simulink model "commhdlQPSKTxRxLoopback"  (R2025b)
settings: Solver=FixedStepDiscrete  StartTime=0.0  StopTime=stopTime  RelTol=1e-3
PostLoadFcn:
  | hScopeConfig = get_param([gcs '/Receiver/QPSK Rx/Frequency and Time Synchronizer/Symbol Synchronizer/No HDL/QPSK Receiver Eye Diagram'],'ScopeConfiguration');
  | 
  | hScopeConfig.OpenAtSimulationStart = false;
  | hScopeConfig.Visible = false;
  | SamplesPerSymbol = 4;
  | %UpsamplesRx = 1;
  | clear hScopeConfig
InitFcn:
  | commhdlQPSKTxRxModelInit;
  | % Rate bridge: ADRV9002/Jupiter radio runs at 15.36 MHz = 2x the 7.68 MHz
  | % (4 samples/symbol @ Rsym=1.92 MHz) the QPSK Rx requires. The deployed
  | % Receiver must downsample the ADC stream by 2. UpsamplesRx=1 fed the QPSK
  | % Rx 8 sps (2x-upsampled) and broke symbol sync / the loopback bit check.
  | UpsamplesRx = 1;   %% T8 RATE FIX: rail 15.36e6 == ADC bus rate,
  | %% no ingress decimation (was 2 when the rail sat on the 7.68e6 rung)
  | UpsamplesTx = 1;
  | clear simTimingOffset;
StopFcn:
  | if exist('simTimingOffset','var')
  |   disp('Simulation completed');
  |   %QPSKTxRxVerification;
  | end
undefined symbols (not defined in the file or in its folder): Add, Config, fsym, randsrc, RandStream, Rsym, Shift
libraries: hdlsllib x141, simulink x43, dspsigops x34, dsphdlfiltering2 x6, dsphdlsigops2 x4, dsphdlmathfun2 x4, commdigbbndpm3 x4, dspmlti4 x2, commchan3 x1, commrflib2 x1, commcnvcod2 x1
(part 2 of 8)

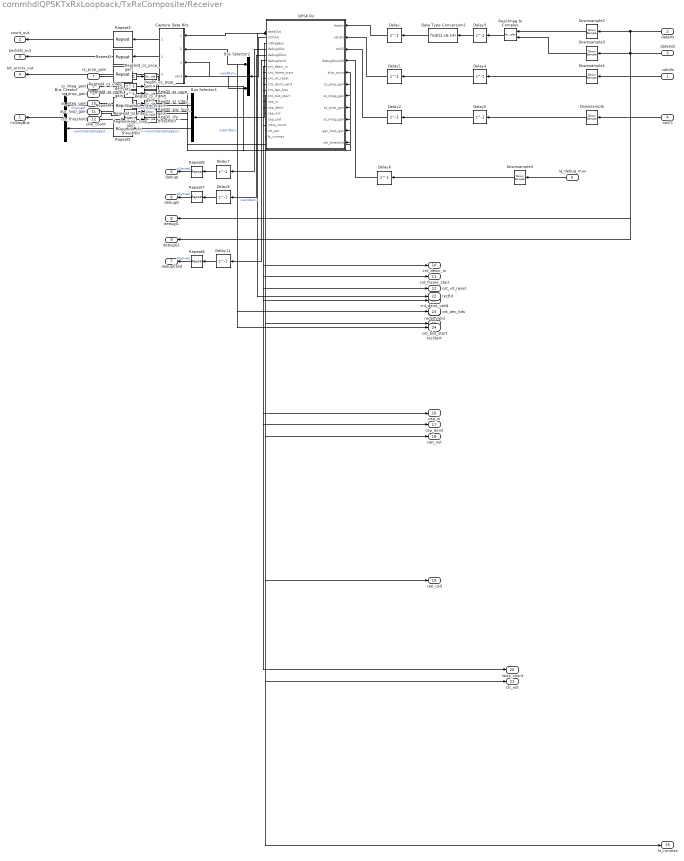
== system commhdlQPSKTxRxLoopback/TxRxComposite/Receiver ==
  validIn : Inport
  dataInI : Inport  Port=2
  dataInQ : Inport  Port=3
  rstCS : Inport  Port=4
  iq_debug_mux : Inport  Port=5  OutDataTypeStr=uint32
  skip_count : Inport  Port=6  OutDataTypeStr=uint32  SampleTime=1/15.36e6
  cs_prop_gain : Inport  Port=7  OutDataTypeStr=uint32  SampleTime=1/15.36e6
  cs_integ_gain : Inport  Port=8  OutDataTypeStr=uint32  SampleTime=1/15.36e6
  ss_prop_gain : Inport  Port=9  OutDataTypeStr=uint32  SampleTime=1/15.36e6
  ss_integ_gain : Inport  Port=10  OutDataTypeStr=uint32  SampleTime=1/15.36e6
  agc_loop_gain : Inport  Port=11  OutDataTypeStr=uint32  SampleTime=1/15.36e6
  cfo_threshold : Inport  Port=12  OutDataTypeStr=uint32  SampleTime=1/15.36e6
  Bus Creator : BusCreator  Inputs=2
  Bus Selector1 : BusSelector  OutputSignals=nSynced,normCoarseFreqEst
  Bus Selector2 : BusSelector  OutputSignals=startOut,endOut,validOut
  Capture Data Bits : Subsystem
  Data Type Conversion2 : DataTypeConversion  OutDataTypeStr=fixdt(1,16,14)  ConvertRealWorld=Stored Integer (SI)  SaturateOnIntegerOverflow=off  RndMeth=Floor
  Delay{,1..8,11} (10 alike) : Delay  DelayLength=1
  Downsample{,1..4} (5 alike) : DownSample  N=UpsamplesRx  RateOptions=Allow multirate processing
  QPSK Rx : Subsystem
      mask init: same as commhdlQPSKTxRxLoopback/Receiver/QPSK Rx
  Real-Imag to Complex : RealImagToComplex
  RegDS_agc_loop_gain : DownSample  N=1  RateOptions=Allow multirate processing  AllowArbitraryFixedInput=on
  RegDS_cfo_threshold : DownSample  N=1  RateOptions=Allow multirate processing  AllowArbitraryFixedInput=on
  RegDS_cs_integ_gain : DownSample  N=1  RateOptions=Allow multirate processing  AllowArbitraryFixedInput=on
  RegDS_cs_prop_gain : DownSample  N=1  RateOptions=Allow multirate processing  AllowArbitraryFixedInput=on
  RegDS_ss_integ_gain : DownSample  N=1  RateOptions=Allow multirate processing  AllowArbitraryFixedInput=on
  RegDS_ss_prop_gain : DownSample  N=1  RateOptions=Allow multirate processing  AllowArbitraryFixedInput=on
  RegHold_agc_loop_gain : Delay  DelayLength=1
  RegHold_cfo_threshold : Delay  DelayLength=1
  RegHold_cs_integ_gain : Delay  DelayLength=1
  RegHold_cs_prop_gain : Delay  DelayLength=1
  RegHold_ss_integ_gain : Delay  DelayLength=1
  RegHold_ss_prop_gain : Delay  DelayLength=1
  Repeat{1..8} (8 alike) : dspsigops/Repeat  FactorSource=Dialog parameter  N=UpsamplesRx  Nmax=16  InputProcessing=Columns as channels (frame based)  RateOptions=Allow multirate processing  ic=0  mode=Unused parameter value
      settings: LibrarySourceBlock=commsequence2/Repeat
  SkipDS : DownSample  N=1  RateOptions=Allow multirate processing  AllowArbitraryFixedInput=on
  SkipHold : Delay  DelayLength=1
  rxDiagBus : Outport
  count_out : Outport  Port=2
  packets_out : Outport  Port=3
  bit_errors_out : Outport  Port=4
  debugI : Outport  Port=5
  debugQ : Outport  Port=6
  debugValid : Outport  Port=7
  debugI1 : Outport  Port=8
  debugQ1 : Outport  Port=9
  cnt_descr_in : Outport  Port=10
  cnt_frame_start : Outport  Port=11
  cnt_vit_reset : Outport  Port=12
  cnt_deint_valid : Outport  Port=13
  cnt_dec_bits : Outport  Port=14
  cnt_bist_start : Outport  Port=15
  cap_in : Outport  Port=16
  cap_deint : Outport  Port=17
  cap_out : Outport  Port=18
  cap_cad : Outport  Port=19
  rstcs_count : Outport  Port=20
  cfc_est : Outport  Port=21
  recBit : Outport  Port=22
  recBitValid : Outport  Port=23
  recStart : Outport  Port=24
  fs_runmax : Outport  Port=25
  wires:
  Downsample/1 -> Delay5/1
  Delay11/1 -> Repeat8/1
  Delay8/1 -> Repeat7/1
  Delay7/1 -> Repeat6/1
  QPSK Rx/6(debugValid) -> Delay11/1
  Repeat8/1 -> debugValid/1  "nSynced"
  Downsample4/1 -> Delay6/1
  Delay6/1 -> QPSK Rx/4(debugMuxCtrl)
  iq_debug_mux/1 -> Downsample4/1
  Repeat7/1 -> debugQ/1  "nSynced"
  Repeat6/1 -> debugI/1  "nSynced"
  QPSK Rx/5(debugQOut) -> Delay8/1
  QPSK Rx/4(debugIOut) -> Delay7/1
  Delay5/1 -> Delay2/1
  Delay4/1 -> Delay1/1
  Delay3/1 -> Data Type Conversion2/1
  Delay2/1 -> QPSK Rx/3(rstCS)
  Delay1/1 -> QPSK Rx/2(validIn)
  Delay/1 -> QPSK Rx/1(dataIn)
  Data Type Conversion2/1 -> Delay/1
  Downsample3/1 -> Real-Imag to Complex/2
  Downsample2/1 -> Real-Imag to Complex/1
  Real-Imag to Complex/1 -> Delay3/1
  dataInI/1 -> Downsample2/1, debugI1/1
  dataInQ/1 -> Downsample3/1, debugQ1/1
  Repeat5/1 -> Bus Creator/2  "normCoarseFreqEst"
  Repeat4/1 -> Bus Creator/1  "nSynced"
  Bus Selector1/2 -> Repeat5/1  "<normCoarseFreqEst>"
  Bus Selector1/1 -> Repeat4/1  "<nSynced>"
  Bus Creator/1 -> rxDiagBus/1
  QPSK Rx/3(rxDiagBus) -> Bus Selector1/1
  Repeat3/1 -> count_out/1
  Repeat2/1 -> packets_out/1
  Repeat1/1 -> bit_errors_out/1
  Downsample1/1 -> Delay4/1
  Capture Data Bits/3(bit_errors_out) -> Repeat1/1
  Capture Data Bits/2(packets_out) -> Repeat2/1
  Capture Data Bits/1(count_out) -> Repeat3/1
  Bus Selector2/3 -> Capture Data Bits/4(valid), recBitValid/1  "<validOut>"
  validIn/1 -> Downsample1/1
  rstCS/1 -> Downsample/1
  Bus Selector2/2 -> Capture Data Bits/3(dataEnd)  "<endOut>"
  QPSK Rx/2(ctrlOut) -> Bus Selector2/1
  QPSK Rx/1(dataOut) -> Capture Data Bits/1(dataOut), recBit/1
  Bus Selector2/1 -> Capture Data Bits/2(dataSrt), recStart/1  "<startOut>"
  QPSK Rx/7(cnt_descr_in) -> cnt_descr_in/1
  QPSK Rx/8(cnt_frame_start) -> cnt_frame_start/1
  QPSK Rx/9(cnt_vit_reset) -> cnt_vit_reset/1
  QPSK Rx/10(cnt_deint_valid) -> cnt_deint_valid/1
  QPSK Rx/11(cnt_dec_bits) -> cnt_dec_bits/1
  QPSK Rx/12(cnt_bist_start) -> cnt_bist_start/1
  skip_count/1 -> SkipHold/1
  SkipHold/1 -> SkipDS/1
  SkipDS/1 -> QPSK Rx/5(skip_count)
  QPSK Rx/13(cap_in) -> cap_in/1
  QPSK Rx/14(cap_deint) -> cap_deint/1
  QPSK Rx/15(cap_out) -> cap_out/1
  QPSK Rx/16(cap_cad) -> cap_cad/1
  QPSK Rx/17(rstcs_count) -> rstcs_count/1
  QPSK Rx/18(cfc_est) -> cfc_est/1
  cs_prop_gain/1 -> RegHold_cs_prop_gain/1
  RegHold_cs_prop_gain/1 -> RegDS_cs_prop_gain/1
  RegDS_cs_prop_gain/1 -> QPSK Rx/6(cs_prop_gain)
  cs_integ_gain/1 -> RegHold_cs_integ_gain/1
  RegHold_cs_integ_gain/1 -> RegDS_cs_integ_gain/1
  RegDS_cs_integ_gain/1 -> QPSK Rx/7(cs_integ_gain)
  ss_prop_gain/1 -> RegHold_ss_prop_gain/1
  RegHold_ss_prop_gain/1 -> RegDS_ss_prop_gain/1
  RegDS_ss_prop_gain/1 -> QPSK Rx/8(ss_prop_gain)
  ss_integ_gain/1 -> RegHold_ss_integ_gain/1
  RegHold_ss_integ_gain/1 -> RegDS_ss_integ_gain/1
  RegDS_ss_integ_gain/1 -> QPSK Rx/9(ss_integ_gain)
  agc_loop_gain/1 -> RegHold_agc_loop_gain/1
  RegHold_agc_loop_gain/1 -> RegDS_agc_loop_gain/1
  RegDS_agc_loop_gain/1 -> QPSK Rx/10(agc_loop_gain)
  cfo_threshold/1 -> RegHold_cfo_threshold/1
  RegHold_cfo_threshold/1 -> RegDS_cfo_threshold/1
  RegDS_cfo_threshold/1 -> QPSK Rx/11(cfo_threshold)
  QPSK Rx/19(fs_runmax) -> fs_runmax/1

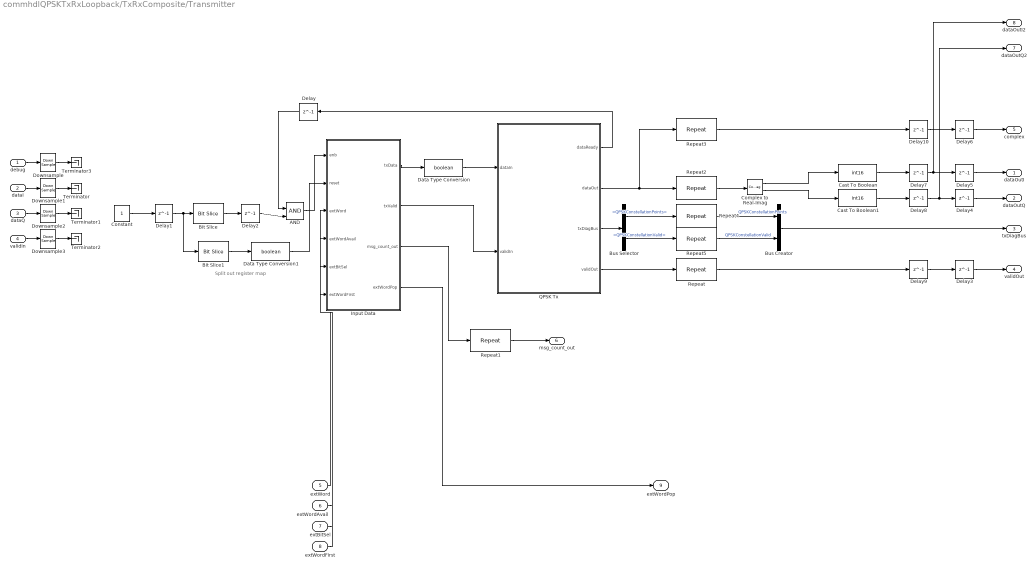
== system commhdlQPSKTxRxLoopback/TxRxComposite/Transmitter ==
  note: Split out register map
  debug : Inport  PortDimensions=1
  dataI : Inport  Port=2
  dataQ : Inport  Port=3
  validIn : Inport  Port=4
  extWord : Inport  Port=5  OutDataTypeStr=uint64
  extWordAvail : Inport  Port=6  OutDataTypeStr=boolean
  extBitSel : Inport  Port=7  OutDataTypeStr=boolean
  extWordFirst : Inport  Port=8  OutDataTypeStr=boolean
  AND : Logic  IconShape=distinctive  AllPortsSameDT=off  OutDataTypeStr=boolean
  Bit Slice : hdlsllib/Logic and Bit Operations/Bit Slice  lidx=0  ridx=0
  Bit Slice1 : hdlsllib/Logic and Bit Operations/Bit Slice  lidx=1  ridx=1
  Bus Creator : BusCreator  Inputs=2
  Bus Selector : BusSelector  OutputSignals=QPSKConstellationPoints,QPSKConstellationValid
  Cast To Boolean : DataTypeConversion  OutDataTypeStr=int16  ConvertRealWorld=Stored Integer (SI)  SaturateOnIntegerOverflow=off  RndMeth=Floor
  Cast To Boolean1 : DataTypeConversion  OutDataTypeStr=int16  ConvertRealWorld=Stored Integer (SI)  SaturateOnIntegerOverflow=off  RndMeth=Floor
  Complex to Real-Imag : ComplexToRealImag
  Constant : Constant  OutDataTypeStr=uint32  SampleTime=-1
  Data Type Conversion : DataTypeConversion  OutDataTypeStr=boolean  SaturateOnIntegerOverflow=off  RndMeth=Floor
  Data Type Conversion1 : DataTypeConversion  OutDataTypeStr=boolean  SaturateOnIntegerOverflow=off  RndMeth=Floor
  Delay{,1..10} (11 alike) : Delay  DelayLength=1
  Downsample{,1..3} (4 alike) : DownSample  N=UpsamplesTx  RateOptions=Allow multirate processing
  Input Data : Subsystem  mask{dataBits=reshape(repmat(randsrc(2240*1,1,[0,1],RandStream('mcg16807','Seed',0)), 59,1), [2240*59,1]), Rsym=3.84e6}
      mask prompts: dataBits "Data Bits :"; Rsym "Symbol Rate (in baud rate)  :"
      mask Display: disp(['Double-Click' newline 'to set data bits']);
  QPSK Tx : Subsystem
      mask init: same as commhdlQPSKTxRxLoopback/Transmitter/QPSK Tx
  Repeat{,1..5} (6 alike) : dspsigops/Repeat  FactorSource=Dialog parameter  N=UpsamplesTx  Nmax=16  InputProcessing=Columns as channels (frame based)  RateOptions=Allow multirate processing  ic=0  mode=Unused parameter value
      settings: LibrarySourceBlock=commsequence2/Repeat
  Terminator{,1..3} (4 alike) : Terminator
  dataOutI : Outport
  dataOutQ : Outport  Port=2
  txDiagBus : Outport  Port=3
  validOut : Outport  Port=4
  complex : Outport  Port=5
  msg_count_out : Outport  Port=6
  dataOutQ2 : Outport  Port=7
  dataOutI2 : Outport  Port=8
  extWordPop : Outport  Port=9
  wires:
  Delay10/1 -> Delay6/1
  Delay9/1 -> Delay3/1
  Delay8/1 -> Delay4/1, dataOutQ2/1
  Delay7/1 -> Delay5/1, dataOutI2/1
  Delay6/1 -> complex/1
  Delay5/1 -> dataOutI/1
  Delay4/1 -> dataOutQ/1
  Delay3/1 -> validOut/1
  Cast To Boolean1/1 -> Delay8/1
  Cast To Boolean/1 -> Delay7/1
  Bus Creator/1 -> txDiagBus/1
  Repeat5/1 -> Bus Creator/2  "QPSKConstellationValid"
  Bus Selector/2 -> Repeat5/1  "<QPSKConstellationValid>"
  Repeat4/1 -> Bus Creator/1  "QPSKConstellationPoints"
  Bus Selector/1 -> Repeat4/1  "<QPSKConstellationPoints>"
  QPSK Tx/3(txDiagBus) -> Bus Selector/1
  Repeat1/1 -> msg_count_out/1
  Downsample3/1 -> Terminator2/1
  Downsample2/1 -> Terminator1/1
  Downsample1/1 -> Terminator/1
  Downsample/1 -> Terminator3/1
  Repeat3/1 -> Delay10/1
  Repeat2/1 -> Complex to Real-Imag/1
  Repeat/1 -> Delay9/1
  Input Data/3(msg_count_out) -> Repeat1/1
  Complex to Real-Imag/2 -> Cast To Boolean1/1
  Complex to Real-Imag/1 -> Cast To Boolean/1
  QPSK Tx/2(dataOut) -> Repeat2/1, Repeat3/1
  debug/1 -> Downsample/1
  Constant/1 -> Delay1/1
  validIn/1 -> Downsample3/1
  dataQ/1 -> Downsample2/1
  dataI/1 -> Downsample1/1
  Data Type Conversion1/1 -> Input Data/2(reset)
  Bit Slice1/1 -> Data Type Conversion1/1
  Delay2/1 -> AND/2
  Delay1/1 -> Bit Slice/1, Bit Slice1/1
  Delay/1 -> AND/1
  Bit Slice/1 -> Delay2/1
  AND/1 -> Input Data/1(enb)
  QPSK Tx/1(dataReady) -> Delay/1
  QPSK Tx/4(validOut) -> Repeat/1
  Data Type Conversion/1 -> QPSK Tx/1(dataIn)
  Input Data/1(txData) -> Data Type Conversion/1
  Input Data/2(txValid) -> QPSK Tx/2(validIn)
  extWord/1 -> Input Data/3(extWord)
  extWordAvail/1 -> Input Data/4(extWordAvail)
  extBitSel/1 -> Input Data/5(extBitSel)
  extWordFirst/1 -> Input Data/6(extWordFirst)
  Input Data/4(extWordPop) -> extWordPop/1

== system commhdlQPSKTxRxLoopback/Receiver/QPSK Rx/Automatic Gain Control ==
  dataIn : Inport
  validIn : Inport  Port=2
  Data Type Conversion : DataTypeConversion  OutDataTypeStr=fixdt(1,16,10)  SaturateOnIntegerOverflow=off  RndMeth=Floor
  Delay{1..5} (5 alike) : Delay
  Error Detector : Subsystem
  Loop Filter : Subsystem
  Product : Product  OutDataTypeStr=Inherit: Same as first input
  dataOut : Outport
  validOut : Outport  Port=2
  wires:
  Data Type Conversion/1 -> Delay1/1
  Delay5/1 -> Delay3/1
  Delay3/1 -> validOut/1
  Delay4/1 -> Product/1
  Delay1/1 -> Product/2
  Loop Filter/1(gain) -> Data Type Conversion/1
  Error Detector/1(err) -> Loop Filter/1(err)
  validIn/1 -> Delay5/1
  Delay2/1 -> Error Detector/1(dataIn), dataOut/1
  dataIn/1 -> Delay4/1
  Product/1 -> Delay2/1

== system commhdlQPSKTxRxLoopback/Receiver/QPSK Rx/Frequency and Time Synchronizer ==
  dataIn : Inport
  validIn : Inport  Port=2
  rstCS : Inport  Port=3
  Carrier Synchronizer : Subsystem
      settings: PortSchema="{\"entries\":[{\"content\":{\"sides\":[{\"content\":{\"connectorIds\":[\"In1\",\"In2\",\"In3\"]},\"type\":\"ConnectorPlacement.EquallySpacedRectSide\",\"uuid\":\"ee58e5dc-083a-48cb-b7f3-66ed8a15890f\"},{\"content\":{\"connectorIds\":[\"Out1\",\"Out2\"],\"side\":\"RIGHT\"},\"type\":\"ConnectorPlacement.EquallySpacedRectSide\",\"uuid\":\"6d121164-5065-4840-a82e-fa57a8e9650e\"},{\"content\":{\"connectorIds\":[\"In4\"],\"side\":\"TOP\"},\"type\":\"ConnectorPlacement.EquallySpacedRectSide\",\"uuid\":\"54d2b8e3-f516-4572-94a0-c914196ae8e4\"}]},\"type\":\"ConnectorPlacement.EquallySpacedConnector\",\"uuid\":\"0f2a6472-efd0-42ca-a030-ab436081b5e1\"}],\"packageUris\":[\"http://schema.mathworks.com/mf0/Connector/R2020b\"],\"version\":\"1.0\"}"
  Coarse Frequency Compensator : Subsystem
      settings: PortSchema="{\"entries\":[{\"content\":{\"sides\":[{\"content\":{\"connectorIds\":[\"In1\",\"In2\"]},\"type\":\"ConnectorPlacement.EquallySpacedRectSide\",\"uuid\":\"138aa5bd-62db-47d6-b55f-f529a6004434\"},{\"content\":{\"connectorIds\":[\"Out1\",\"Out2\",\"Out3\"],\"side\":\"RIGHT\"},\"type\":\"ConnectorPlacement.EquallySpacedRectSide\",\"uuid\":\"8e6ccec0-f736-48ab-be6d-feac886e083d\"},{\"content\":{\"connectorIds\":[\"Out4\"],\"side\":\"TOP\"},\"type\":\"ConnectorPlacement.EquallySpacedRectSide\",\"uuid\":\"d4535392-74fa-432a-a39c-b98ba26e8163\"},{\"content\":{\"side\":\"BOTTOM\"},\"type\":\"ConnectorPlacement.EquallySpacedRectSide\",\"uuid\":\"770ac6a2-7a02-4a77-858b-592982deaf6e\"}]},\"type\":\"ConnectorPlacement.EquallySpacedConnector\",\"uuid\":\"a9b944be-f88b-4ab6-a5e1-6824362eb9ca\"}],\"packageUris\":[\"http://schema.mathworks.com/mf0/Connector/R2020b\"],\"version\":\"1.0\"}"
  No HDL : Subsystem
      settings: PortSchema="{\"entries\":[{\"content\":{\"sides\":[{\"content\":{\"connectorIds\":[\"In1\",\"In2\"]},\"type\":\"ConnectorPlacement.EquallySpacedRectSide\",\"uuid\":\"df96a46d-149f-4580-adf6-e5cf26cffa9b\"},{\"content\":{\"connectorIds\":[\"In3\",\"In4\"],\"side\":\"RIGHT\"},\"type\":\"ConnectorPlacement.EquallySpacedRectSide\",\"uuid\":\"1c46d09c-cb37-4618-ac4e-e5ef50df41fb\"},{\"content\":{\"connectorIds\":[],\"side\":\"TOP\"},\"type\":\"ConnectorPlacement.EquallySpacedRectSide\",\"uuid\":\"7fe62300-46d7-4234-a31d-eecffed4f6e6\"},{\"content\":{\"connectorIds\":[],\"side\":\"BOTTOM\"},\"type\":\"ConnectorPlacement.EquallySpacedRectSide\",\"uuid\":\"05ecd563-28f5-4cfd-b718-5032a7458763\"}]},\"type\":\"ConnectorPlacement.EquallySpacedConnector\",\"uuid\":\"4b3d5859-a469-4389-9e5d-e5f07416a9a1\"}],\"packageUris\":[\"http://schema.mathworks.com/mf0/Connector/R2020b\"],\"version\":\"1.0\"}"
  Packet Controller : Subsystem
  Phase Ambiguity Estimation and Correction : Subsystem
  Preamble Detector : Subsystem
  Symbol Synchronizer : Subsystem
  dataOut : Outport
  startOut : Outport  Port=2
  endOut : Outport  Port=3
  validOut : Outport  Port=4
  postSymbolSync : Outport  Port=5
  postCarrierSync : Outport  Port=6
  nSynced : Outport  Port=7
  normCoarseFreqEst : Outport  Port=8
  wires:
  Coarse Frequency Compensator/3(validOut) -> Carrier Synchronizer/3(validIn)
  Coarse Frequency Compensator/1(dataOut) -> Carrier Synchronizer/1(dataIn)
  Phase Ambiguity Estimation and Correction/1(dataOut) -> Packet Controller/1(dataIn)
  Phase Ambiguity Estimation and Correction/3(validOut) -> Packet Controller/3(validIn)
  Symbol Synchronizer/2(validOut) -> No HDL/2(In2), Coarse Frequency Compensator/2(validIn)
  Symbol Synchronizer/1(dataOut) -> postSymbolSync/1, No HDL/1(In1), Coarse Frequency Compensator/1(dataIn)
  Phase Ambiguity Estimation and Correction/2(syncPulseOut) -> Packet Controller/2(syncPulse)
  Preamble Detector/3(validOut) -> Phase Ambiguity Estimation and Correction/3(validIn)
  Preamble Detector/1(dataOut) -> Phase Ambiguity Estimation and Correction/1(dataIn)
  validIn/1 -> Symbol Synchronizer/2(validIn)
  dataIn/1 -> Symbol Synchronizer/1(dataIn)
  Coarse Frequency Compensator/2(rstCS) -> Carrier Synchronizer/2(internalRst)
  Packet Controller/1(dataOut) -> dataOut/1
  Packet Controller/2(startOut) -> startOut/1
  Packet Controller/3(endOut) -> endOut/1
  Packet Controller/4(validOut) -> validOut/1
  Preamble Detector/2(syncPulse) -> nSynced/1, Phase Ambiguity Estimation and Correction/2(syncPulseIn)
  Carrier Synchronizer/1(dataOut) -> postCarrierSync/1, No HDL/3(In3), Preamble Detector/1(dataIn)
  Carrier Synchronizer/2(validOut) -> No HDL/4(In4), Preamble Detector/2(validIn)
  Coarse Frequency Compensator/4(normalizedFreqEst) -> normCoarseFreqEst/1
  rstCS/1 -> Carrier Synchronizer/4(manualRst)

== system commhdlQPSKTxRxLoopback/Receiver/QPSK Rx/HDL Data Descrambler ==
  note: HDL Data Scrambler
      | Polynomial: x^7+x^4+1
      | Initial state: [1 0 1 1 1 0 1]
  dataIn : Inport
  startIn : Inport  Port=2
  endIn : Inport  Port=3
  validIn : Inport  Port=4
  BIT_XOR : Logic  Operator=XOR  IconShape=distinctive  AllPortsSameDT=off  OutDataTypeStr=boolean
  BIT_XOR2 : Logic  Operator=XOR  IconShape=distinctive  AllPortsSameDT=off  OutDataTypeStr=boolean
  Delay{,1..7} (8 alike) : Delay  DelayLength=1
  EnableScrambling : Constant  Value=true  SampleTime=-1
  Logical Operator : Logic  IconShape=distinctive  AllPortsSameDT=off  OutDataTypeStr=boolean
  Switch : Switch  Criteria=u2 > Threshold  SaturateOnIntegerOverflow=off  InputSameDT=off
  Unit Delay Enabled Resettable Synchronous{,2..3,5,7} (5 alike) : hdlsllib/Discrete/Unit Delay Enabled Resettable Synchronous  InitialCondition=1  SampleTime=-1
  Unit Delay Enabled Resettable Synchronous1 : hdlsllib/Discrete/Unit Delay Enabled Resettable Synchronous  InitialCondition=0  SampleTime=-1
  Unit Delay Enabled Resettable Synchronous4 : hdlsllib/Discrete/Unit Delay Enabled Resettable Synchronous  InitialCondition=0  SampleTime=-1
  Unit Delay Enabled Resettable Synchronous6 : hdlsllib/Discrete/Unit Delay Enabled Resettable Synchronous  InitialCondition=0.0  SampleTime=-1
  dataOut : Outport  InitialOutput=0
  startOut : Outport  Port=2  InitialOutput=0
  endOut : Outport  Port=3  InitialOutput=0
  validOut : Outport  Port=4  InitialOutput=0
  wires:
  Delay4/1 -> validOut/1
  Delay3/1 -> dataOut/1
  endIn/1 -> Delay2/1, Unit Delay Enabled Resettable Synchronous4/3
  Logical Operator/1 -> BIT_XOR2/2
  Unit Delay Enabled Resettable Synchronous4/1 -> Logical Operator/1
  Delay1/1 -> Unit Delay Enabled Resettable Synchronous6/2, Unit Delay Enabled Resettable Synchronous2/2, Unit Delay Enabled Resettable Synchronous1/2, Unit Delay Enabled Resettable Synchronous/2, Delay4/1, Unit Delay Enabled Resettable Synchronous3/2, Unit Delay Enabled Resettable Synchronous5/2, Unit Delay Enabled Resettable Synchronous7/2
  Delay/1 -> Switch/3, BIT_XOR2/1
  startIn/1 -> Delay5/1, Unit Delay Enabled Resettable Synchronous4/1, Unit Delay Enabled Resettable Synchronous4/2, Unit Delay Enabled Resettable Synchronous6/3, Unit Delay Enabled Resettable Synchronous5/3, Unit Delay Enabled Resettable Synchronous1/3, Unit Delay Enabled Resettable Synchronous/3, Unit Delay Enabled Resettable Synchronous2/3, Unit Delay Enabled Resettable Synchronous3/3, Unit Delay Enabled Resettable Synchronous7/3
  dataIn/1 -> Delay/1
  validIn/1 -> Delay1/1
  BIT_XOR/1 -> Unit Delay Enabled Resettable Synchronous/1, Logical Operator/2
  Unit Delay Enabled Resettable Synchronous1/1 -> Unit Delay Enabled Resettable Synchronous2/1
  Unit Delay Enabled Resettable Synchronous2/1 -> Unit Delay Enabled Resettable Synchronous3/1
  Unit Delay Enabled Resettable Synchronous/1 -> Unit Delay Enabled Resettable Synchronous1/1
  Unit Delay Enabled Resettable Synchronous3/1 -> BIT_XOR/2, Unit Delay Enabled Resettable Synchronous5/1
  Unit Delay Enabled Resettable Synchronous5/1 -> Unit Delay Enabled Resettable Synchronous6/1
  Unit Delay Enabled Resettable Synchronous6/1 -> Unit Delay Enabled Resettable Synchronous7/1
  Unit Delay Enabled Resettable Synchronous7/1 -> BIT_XOR/1
  Delay2/1 -> Delay6/1
  Delay5/1 -> Delay7/1
  Delay6/1 -> endOut/1
  Delay7/1 -> startOut/1
  EnableScrambling/1 -> Switch/2
  BIT_XOR2/1 -> Switch/1
  Switch/1 -> Delay3/1

== system commhdlQPSKTxRxLoopback/Receiver/QPSK Rx/QPSK Demodulator ==
  dataIn : Inport
  startIn : Inport  Port=2
  endIn : Inport  Port=3
  validIn : Inport  Port=4
  Delay{,1..13} (14 alike) : Delay  DelayLength=1
  QPSK Demodulator Baseband : commdigbbndpm3/QPSK Demodulator Baseband  OutType=Bit  DecType=Hard decision  VarSource=Dialog  Variance=1  Dec=Gray  Ph=pi/4  outDtype1=boolean  outDtype2=Inherit via internal rule  derotateFactorWordLen=16  derotateFactorDataTypeStr=Inherit: Same word length as input  derotateFactorLastDataTypeStr=Inherit: Same word length as input
  Serializer : Subsystem
  Signal Specification : SignalSpecification  Dimensions=1
  dataOut : Outport
  startOut : Outport  Port=2
  endOut : Outport  Port=3
  validOut : Outport  Port=4
  wires:
  Delay/1 -> QPSK Demodulator Baseband/1
  Delay1/1 -> Delay5/1
  Delay6/1 -> Delay4/1
  Delay7/1 -> Delay13/1
  Delay2/1 -> Delay6/1
  Delay3/1 -> Delay7/1
  Signal Specification/1 -> Delay/1
  QPSK Demodulator Baseband/1 -> Delay12/1
  Delay8/1 -> dataOut/1
  Delay9/1 -> validOut/1
  Delay10/1 -> startOut/1
  Delay11/1 -> endOut/1
  Delay5/1 -> Serializer/2(In2)
  Delay12/1 -> Serializer/1(u)
  Delay4/1 -> Delay10/1
  Delay13/1 -> Delay11/1
  Serializer/1(Out1) -> Delay8/1
  Serializer/2(Out2) -> Delay9/1
  dataIn/1 -> Signal Specification/1
  validIn/1 -> Delay1/1
  startIn/1 -> Delay2/1
  endIn/1 -> Delay3/1

== system commhdlQPSKTxRxLoopback/Transmitter/Input Data/Message Generator ==
  reset : Inport
  enable : Inport  Port=2
  MATLAB Function : MATLAB Function  TreatAsAtomicUnit=on
  out : Outport
  stop : Outport  Port=2
  start : Outport  Port=3
  valid : Outport  Port=4
  count : Outport  Port=5
  msg_count_out : Outport  Port=6
  wires:
  MATLAB Function/3(stop) -> stop/1
  MATLAB Function/1(out) -> out/1
  reset/1 -> MATLAB Function/2(reset)
  MATLAB Function/2(start) -> start/1
  enable/1 -> MATLAB Function/1(enable)
  MATLAB Function/4(valid) -> valid/1
  MATLAB Function/5(count_out) -> count/1
  MATLAB Function/6(msg_count_out) -> msg_count_out/1

== system commhdlQPSKTxRxLoopback/Transmitter/QPSK Tx/Bit Packetizer ==
  dataIn : Inport
  validIn : Inport  Port=2
  Compare To Constant : hdlsllib/Logic and Bit Operations/Compare To Constant  relop===  const=length(Preamble)  OutDataTypeStr=boolean
  Compare To Constant1 : hdlsllib/Logic and Bit Operations/Compare To Constant  relop===  const=bitsPerPacket - 1  OutDataTypeStr=boolean
  Compare To Constant2 : hdlsllib/Logic and Bit Operations/Compare To Constant  relop=>=  const=length(Preamble)  OutDataTypeStr=boolean
  Data Bits FIFO : Subsystem
  Data Type Conversion : DataTypeConversion  OutDataTypeStr=boolean  SaturateOnIntegerOverflow=off  RndMeth=Floor
  DataReadyPaceCmp : simulink/Logic and Bit Operations/Compare To Constant  relop===  const=SamplesPerSymbol/2 - 1  OutDataTypeStr=boolean
  HDL Counter : hdlsllib/Sources/HDL Counter  CountType=Count limited  CountInit=0  CountStep=1  CountMax=SamplesPerSymbol/2 - 1  CountFromType=Initial value  CountFrom=0  CountResetPort=off  CountLoadPort=off  CountEnbPort=on  CountDirPort=off  CountHitOutputPort=off  CountDataType=Unsigned  CountWordLen=nextpow2(SamplesPerSymbol/2)  CountFracLen=0  CountSampTime=1
  Logical Operator : Logic  AllPortsSameDT=off  OutDataTypeStr=boolean
  Logical Operator1 : Logic  AllPortsSameDT=off  OutDataTypeStr=boolean
  Logical Operator2 : Logic  Operator=NOT  AllPortsSameDT=off  OutDataTypeStr=boolean
  Preamble Bits Generator : Subsystem
  Switch : Switch  Criteria=u2 ~= 0  SaturateOnIntegerOverflow=off  InputSameDT=off
  bitsOut : Outport
  dataStart : Outport  Port=2
  dataEnd : Outport  Port=3
  bitsValid : Outport  Port=4
  dataReady : Outport  Port=5
  wires:
  dataIn/1 -> Data Bits FIFO/1(data)
  validIn/1 -> Data Bits FIFO/2(push)
  Compare To Constant/1 -> Logical Operator/1
  Compare To Constant1/1 -> Logical Operator1/2
  Logical Operator/1 -> dataStart/1
  Logical Operator1/1 -> dataEnd/1
  Data Bits FIFO/5(fullRAM) -> Logical Operator2/1
  Logical Operator2/1 -> HDL Counter/1
  Data Bits FIFO/1(dataOut) -> Switch/1
  Data Bits FIFO/3(sampleCount) -> Preamble Bits Generator/2(sampleCount), Compare To Constant/1, Compare To Constant1/1, Compare To Constant2/1
  Data Bits FIFO/4(sampleCountValid) -> bitsValid/1, Logical Operator/2, Logical Operator1/1, Preamble Bits Generator/3(sampleCountValid)
  Data Bits FIFO/2(activeFrame) -> Preamble Bits Generator/1(activeFrame)
  Preamble Bits Generator/1(preambleBits) -> Switch/3
  Compare To Constant2/1 -> Switch/2
  Switch/1 -> bitsOut/1
  Data Type Conversion/1 -> dataReady/1
  HDL Counter/1 -> DataReadyPaceCmp/1
  DataReadyPaceCmp/1 -> Data Type Conversion/1

== system commhdlQPSKTxRxLoopback/Transmitter/QPSK Tx/HDL Data Scrambler ==
  note: HDL Data Scrambler
      | Polynomial: x^7+x^4+1
      | Initial state: [1 0 1 1 1 0 1]
  dataIn : Inport
  startIn : Inport  Port=2
  endIn : Inport  Port=3
  validIn : Inport  Port=4
  BIT_XOR : Logic  Operator=XOR  IconShape=distinctive  AllPortsSameDT=off  OutDataTypeStr=boolean
  BIT_XOR2 : Logic  Operator=XOR  IconShape=distinctive  AllPortsSameDT=off  OutDataTypeStr=boolean
  Delay{,1,3..4} (4 alike) : Delay  DelayLength=1
  EnableScrambling : Constant  Value=true  SampleTime=-1
  Logical Operator : Logic  IconShape=distinctive  AllPortsSameDT=off  OutDataTypeStr=boolean
  Switch : Switch  Criteria=u2 > Threshold  SaturateOnIntegerOverflow=off  InputSameDT=off
  Unit Delay Enabled Resettable Synchronous{,2..3,5,7} (5 alike) : hdlsllib/Discrete/Unit Delay Enabled Resettable Synchronous  InitialCondition=1  SampleTime=-1
  Unit Delay Enabled Resettable Synchronous1 : hdlsllib/Discrete/Unit Delay Enabled Resettable Synchronous  InitialCondition=0  SampleTime=-1
  Unit Delay Enabled Resettable Synchronous4 : hdlsllib/Discrete/Unit Delay Enabled Resettable Synchronous  InitialCondition=0  SampleTime=-1
  Unit Delay Enabled Resettable Synchronous6 : hdlsllib/Discrete/Unit Delay Enabled Resettable Synchronous  InitialCondition=0.0  SampleTime=-1
  dataOut : Outport  InitialOutput=0
  validOut : Outport  Port=2  InitialOutput=0
  wires:
  Delay4/1 -> validOut/1
  Delay3/1 -> dataOut/1
  endIn/1 -> Unit Delay Enabled Resettable Synchronous4/3
  Logical Operator/1 -> BIT_XOR2/2
  Unit Delay Enabled Resettable Synchronous4/1 -> Logical Operator/1
  Delay1/1 -> Unit Delay Enabled Resettable Synchronous6/2, Unit Delay Enabled Resettable Synchronous2/2, Unit Delay Enabled Resettable Synchronous1/2, Unit Delay Enabled Resettable Synchronous/2, Delay4/1, Unit Delay Enabled Resettable Synchronous3/2, Unit Delay Enabled Resettable Synchronous5/2, Unit Delay Enabled Resettable Synchronous7/2
  Delay/1 -> Switch/3, BIT_XOR2/1
  startIn/1 -> Unit Delay Enabled Resettable Synchronous4/1, Unit Delay Enabled Resettable Synchronous4/2, Unit Delay Enabled Resettable Synchronous6/3, Unit Delay Enabled Resettable Synchronous5/3, Unit Delay Enabled Resettable Synchronous1/3, Unit Delay Enabled Resettable Synchronous/3, Unit Delay Enabled Resettable Synchronous2/3, Unit Delay Enabled Resettable Synchronous3/3, Unit Delay Enabled Resettable Synchronous7/3
  dataIn/1 -> Delay/1
  validIn/1 -> Delay1/1
  BIT_XOR/1 -> Unit Delay Enabled Resettable Synchronous/1, Logical Operator/2
  Unit Delay Enabled Resettable Synchronous1/1 -> Unit Delay Enabled Resettable Synchronous2/1
  Unit Delay Enabled Resettable Synchronous2/1 -> Unit Delay Enabled Resettable Synchronous3/1
  Unit Delay Enabled Resettable Synchronous/1 -> Unit Delay Enabled Resettable Synchronous1/1
  Unit Delay Enabled Resettable Synchronous3/1 -> BIT_XOR/2, Unit Delay Enabled Resettable Synchronous5/1
  Unit Delay Enabled Resettable Synchronous5/1 -> Unit Delay Enabled Resettable Synchronous6/1
  Unit Delay Enabled Resettable Synchronous6/1 -> Unit Delay Enabled Resettable Synchronous7/1
  Unit Delay Enabled Resettable Synchronous7/1 -> BIT_XOR/1
  Switch/1 -> Delay3/1
  EnableScrambling/1 -> Switch/2
  BIT_XOR2/1 -> Switch/1

== system commhdlQPSKTxRxLoopback/Transmitter/QPSK Tx/QPSK Modulator ==
  dataIn : Inport
  validIn : Inport  Port=2
  Compare To Constant : simulink/Logic and Bit Operations/Compare To Constant  relop===  const=0  OutDataTypeStr=boolean
  Compare To Constant1 : simulink/Logic and Bit Operations/Compare To Constant  relop===  const=1  OutDataTypeStr=boolean
  Delay{,1..5,11..12} (8 alike) : Delay  DelayLength=1
  HDL Counter : hdlsllib/Sources/HDL Counter  CountType=Count limited  CountInit=0  CountStep=1  CountMax=1  CountFromType=Initial value  CountFrom=0  CountResetPort=off  CountLoadPort=off  CountEnbPort=on  CountDirPort=off  CountHitOutputPort=off  CountDataType=Unsigned  CountWordLen=1  CountFracLen=0  CountSampTime=1
  Logical Operator : Logic  IconShape=distinctive  AllPortsSameDT=off  OutDataTypeStr=boolean
  Logical Operator1 : Logic  IconShape=distinctive  AllPortsSameDT=off  OutDataTypeStr=boolean
  Mux : Mux  Inputs=2
  Null : Constant  Value=complex(0,0)  OutDataTypeStr=fixdt(1,16,15)  SampleTime=1/(Rsym*SamplesPerSymbol)
  QPSK Modulator Baseband : commdigbbndpm3/QPSK Modulator Baseband  InType=Bit  Enc=Gray  Ph=pi/4  outDtype=Fixed-point  outWordLen=16  outUDDataType=sfix(16)  outFracLenMode=User-defined  outFracLen=15  outDataTypeStr=fixdt(1,16,15)  outLastDataTypeStr=fixdt(1,16,15)
  Switch3 : Switch  Threshold=1  SaturateOnIntegerOverflow=off  InputSameDT=off
  Unit Delay Enabled Synchronous : hdlsllib/Discrete/Unit Delay Enabled Synchronous  InitialCondition=0.0  SampleTime=-1
  dataOut : Outport
  validOut : Outport  Port=2
  wires:
  dataIn/1 -> Delay/1
  validIn/1 -> Delay1/1
  HDL Counter/1 -> Compare To Constant/1, Compare To Constant1/1
  QPSK Modulator Baseband/1 -> Delay11/1
  Logical Operator1/1 -> Delay5/1
  Switch3/1 -> Delay2/1
  Null/1 -> Switch3/3
  Delay/1 -> Mux/2, Unit Delay Enabled Synchronous/1
  Delay2/1 -> dataOut/1
  Delay3/1 -> validOut/1
  Delay1/1 -> Logical Operator1/2, Logical Operator/1, HDL Counter/1
  Compare To Constant/1 -> Logical Operator/2
  Compare To Constant1/1 -> Logical Operator1/1
  Delay11/1 -> Switch3/1
  Delay12/1 -> Switch3/2, Delay3/1
  Logical Operator/1 -> Unit Delay Enabled Synchronous/2
  Unit Delay Enabled Synchronous/1 -> Mux/1
  Mux/1 -> Delay4/1
  Delay4/1 -> QPSK Modulator Baseband/1
  Delay5/1 -> Delay12/1

== system commhdlQPSKTxRxLoopback/Transmitter/QPSK Tx/RRC Transmit Filter ==
  dataIn : Inport
  validIn : Inport  Port=2
  Data Type Conversion : DataTypeConversion  OutDataTypeStr=fixdt(1,17,16)  SaturateOnIntegerOverflow=off  RndMeth=Floor
  Data Type Conversion1 : DataTypeConversion  OutDataTypeStr=fixdt(1,16,14)  SaturateOnIntegerOverflow=off  RndMeth=Floor
  Delay1 : Delay  DelayLength=1
  Delay2 : Delay  DelayLength=1
  Delay3 : Delay  DelayLength=1
  RRC Filter : dsphdlfiltering2/Discrete FIR Filter  NumeratorSource=Property  Numerator=RRCCoef  NumeratorPrototype=[]  FilterStructure=Direct form systolic  SerializationOption=Minimum number of cycles between valid input samples  NumCycles=2  NumberOfMultipliers=2  SimulateUsing=Code generation  roundingMode=Floor  overflowMode=off  CoefficientsDataTypeStr=Inherit: Same word length as input  OutputDataTypeStr=Inherit: Same word length as input  ResetInputPort=off  HDLGlobalReset=off  CoeffMultiplier=Multiplier  UseMultForPow2Coeff=on  FrameInputSymmOptim=off
  Unit Delay Enabled Synchronous1 : hdlsllib/Discrete/Unit Delay Enabled Synchronous  InitialCondition=0  SampleTime=-1
  dataOut : Outport
  validOut : Outport  Port=2
  wires:
  dataIn/1 -> Data Type Conversion/1
  RRC Filter/1 -> Data Type Conversion1/1
  RRC Filter/2 -> Delay2/1
  Delay1/1 -> dataOut/1
  Delay2/1 -> validOut/1
  Data Type Conversion/1 -> Delay3/1
  Unit Delay Enabled Synchronous1/1 -> RRC Filter/2
  Data Type Conversion1/1 -> Delay1/1
  validIn/1 -> Unit Delay Enabled Synchronous1/2, Unit Delay Enabled Synchronous1/1
  Delay3/1 -> RRC Filter/1

== system commhdlQPSKTxRxLoopback/TxRxComposite/Receiver/Capture Data Bits ==
  dataOut : Inport
  dataSrt : Inport  Port=2
  dataEnd : Inport  Port=3
  valid : Inport  Port=4
  Display : Display
  Display1 : Display
  Display2 : Display
  MATLAB Function : MATLAB Function  TreatAsAtomicUnit=on
  count_out : Outport
  packets_out : Outport  Port=2
  bit_errors_out : Outport  Port=3
  wires:
  MATLAB Function/3(bit_errors_out) -> Display2/1, bit_errors_out/1
  MATLAB Function/2(packets_out) -> Display1/1, packets_out/1
  MATLAB Function/1(count_out) -> Display/1, count_out/1
  valid/1 -> MATLAB Function/1(valid)
  dataEnd/1 -> MATLAB Function/4(stop)
  dataSrt/1 -> MATLAB Function/3(start)
  dataOut/1 -> MATLAB Function/2(datain)

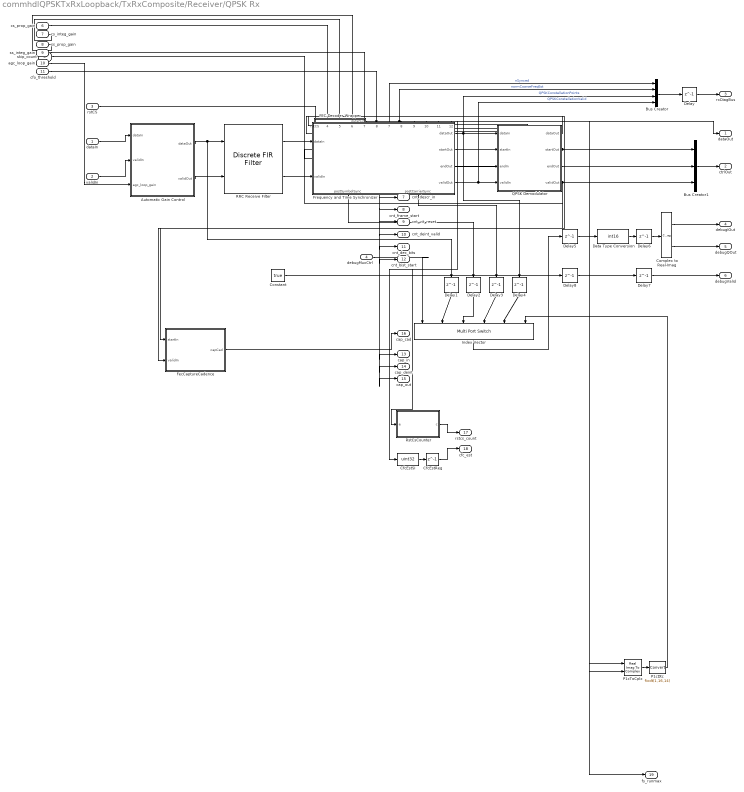
== system commhdlQPSKTxRxLoopback/TxRxComposite/Receiver/QPSK Rx ==
  dataIn : Inport  OutDataTypeStr=fixdt(1,16,14)  PortDimensions=1  SampleTime=1/(Rsym*SamplesPerSymbol)
      settings: SignalType=complex
  validIn : Inport  Port=2  OutDataTypeStr=boolean  PortDimensions=1  SampleTime=1/(Rsym*SamplesPerSymbol)
  rstCS : Inport  Port=3  OutDataTypeStr=boolean  PortDimensions=1
      settings: SignalType=complex
  debugMuxCtrl : Inport  Port=4  OutDataTypeStr=uint32  PortDimensions=1  SampleTime=1/(Rsym*SamplesPerSymbol)
  skip_count : Inport  Port=5  OutDataTypeStr=uint32  SampleTime=1/(Rsym*SamplesPerSymbol)
  cs_prop_gain : Inport  Port=6  OutDataTypeStr=uint32  SampleTime=1/(Rsym*SamplesPerSymbol)
  cs_integ_gain : Inport  Port=7  OutDataTypeStr=uint32  SampleTime=1/(Rsym*SamplesPerSymbol)
  ss_prop_gain : Inport  Port=8  OutDataTypeStr=uint32  SampleTime=1/(Rsym*SamplesPerSymbol)
  ss_integ_gain : Inport  Port=9  OutDataTypeStr=uint32  SampleTime=1/(Rsym*SamplesPerSymbol)
  agc_loop_gain : Inport  Port=10  OutDataTypeStr=uint32  SampleTime=1/(Rsym*SamplesPerSymbol)
  cfo_threshold : Inport  Port=11  OutDataTypeStr=uint32  SampleTime=1/(Rsym*SamplesPerSymbol)
  Automatic Gain Control : Subsystem  mask{Ref=AGCReference, LFG=AGCLoopGain}
      mask prompts: Ref "Error Detector Reference:"; LFG "Loop Filter Gain"
  Bus Creator : BusCreator  Inputs=4
  Bus Creator1 : BusCreator  Inputs=3
  CfcEstReg : Delay  DelayLength=1
  CfcEstSI : DataTypeConversion  OutDataTypeStr=uint32  ConvertRealWorld=Stored Integer (SI)
  Complex to Real-Imag : ComplexToRealImag
  Constant : Constant  Value=true  SampleTime=1/(Rsym*SamplesPerSymbol)
  Data Type Conversion : DataTypeConversion  OutDataTypeStr=int16  ConvertRealWorld=Stored Integer (SI)  SaturateOnIntegerOverflow=off  RndMeth=Floor
  Delay{,1..8} (9 alike) : Delay  DelayLength=1
  FEC Decoder Wrapper : Subsystem
  FecCaptureCadence : MATLAB Function  TreatAsAtomicUnit=on
  Frequency and Time Synchronizer : Subsystem
      settings: PortSchema="{\"entries\":[{\"content\":{\"sides\":[{\"content\":{\"connectorIds\":[\"In1\",\"In2\"]},\"type\":\"ConnectorPlacement.EquallySpacedRectSide\",\"uuid\":\"8bc6a452-5111-4806-8ca9-335cb622aea6\"},{\"content\":{\"connectorIds\":[\"Out1\",\"Out2\",\"Out3\",\"Out4\"],\"side\":\"RIGHT\"},\"type\":\"ConnectorPlacement.EquallySpacedRectSide\",\"uuid\":\"b0f43c98-f5c0-4f62-94ae-d69789942eef\"},{\"content\":{\"connectorIds\":[\"In3\",\"In4\",\"In5\",\"In6\",\"In7\",\"In8\",\"Out7\",\"Out8\",\"Out9\",\"Out10\",\"Out11\",\"Out12\"],\"side\":\"TOP\"},\"type\":\"ConnectorPlacement.EquallySpacedRectSide\",\"uuid\":\"427ff3b3-b896-4008-9584-d311480df763\"},{\"content\":{\"connectorIds\":[\"Out5\",\"Out6\"],\"side\":\"BOTTOM\"},\"type\":\"ConnectorPlacement.EquallySpacedRectSide\",\"uuid\":\"f704cb90-80a1-4198-8b72-e70182b45e73\"},{\"content\":{\"side\":\"HIDDEN\"},\"type\":\"ConnectorPlacement.EquallySpacedRectSide\",\"uuid\":\"f6309498-1e43-486f-b6b5-2c6570711f8e\"}]},\"type\":\"ConnectorPlacement.EquallySpacedConnector\",\"uuid\":\"f0ce492e-c9e1-4b35-98ef-84d77b696cfe\"}],\"packageUris\":[\"http://schema.mathworks.com/mf0/Connector/R2020b\"],\"version\":\"1.0\"}"
  Index Vector : MultiPortSwitch  DataPortOrder=Zero-based contiguous  Inputs=5  DiagnosticForDefault=None  zeroidx=on  SaturateOnIntegerOverflow=off  InputSameDT=off
  P1cDtc : DataTypeConversion  OutDataTypeStr=fixdt(1,16,14)  ConvertRealWorld=Stored Integer (SI)  SaturateOnIntegerOverflow=off  RndMeth=Floor
  P1cToCplx : RealImagToComplex
  QPSK Demodulator : Subsystem
  RRC Receive Filter : dsphdlfiltering2/Discrete FIR Filter  NumeratorSource=Property  Numerator=RRCCoef  NumeratorPrototype=[]  FilterStructure=Direct form systolic  SerializationOption=Minimum number of cycles between valid input samples  NumCycles=2  NumberOfMultipliers=2  SimulateUsing=Code generation  roundingMode=Floor  overflowMode=off  CoefficientsDataTypeStr=Inherit: Same word length as input  OutputDataTypeStr=Inherit: Same word length as input  ResetInputPort=off  HDLGlobalReset=off  CoeffMultiplier=Multiplier  UseMultForPow2Coeff=on  FrameInputSymmOptim=off
  RstCsCounter : MATLAB Function  TreatAsAtomicUnit=on
  dataOut : Outport
  ctrlOut : Outport  Port=2
  rxDiagBus : Outport  Port=3
  debugIOut : Outport  Port=4
  debugQOut : Outport  Port=5
  debugValid : Outport  Port=6
  cnt_descr_in : Outport  Port=7
  cnt_frame_start : Outport  Port=8
  cnt_vit_reset : Outport  Port=9
  cnt_deint_valid : Outport  Port=10
  cnt_dec_bits : Outport  Port=11
  cnt_bist_start : Outport  Port=12
  cap_in : Outport  Port=13
  cap_deint : Outport  Port=14
  cap_out : Outport  Port=15
  cap_cad : Outport  Port=16
  rstcs_count : Outport  Port=17
  cfc_est : Outport  Port=18
  fs_runmax : Outport  Port=19
  wires:
  Constant/1 -> Delay8/1
  Delay8/1 -> Delay7/1
  Delay7/1 -> debugValid/1
  Delay6/1 -> Complex to Real-Imag/1
  Index Vector/1 -> Delay5/1
  Delay5/1 -> Data Type Conversion/1
  Delay4/1 -> Index Vector/5
  Delay3/1 -> Index Vector/4
  Delay2/1 -> Index Vector/3
  Delay1/1 -> Index Vector/2
  Data Type Conversion/1 -> Delay6/1
  Complex to Real-Imag/1 -> debugIOut/1
  Complex to Real-Imag/2 -> debugQOut/1
  debugMuxCtrl/1 -> Index Vector/1
  Frequency and Time Synchronizer/6(postCarrierSync) -> Delay3/1
  Frequency and Time Synchronizer/5(postSymbolSync) -> Delay2/1
  Delay/1 -> rxDiagBus/1
  QPSK Demodulator/4(validOut) -> FecCaptureCadence/2(validIn), FEC Decoder Wrapper/4(validIn)
  Frequency and Time Synchronizer/4(validOut) -> Bus Creator/4, QPSK Demodulator/4(validIn)  "QPSKConstellationValid"
  Frequency and Time Synchronizer/2(startOut) -> QPSK Demodulator/2(startIn)
  QPSK Demodulator/2(startOut) -> FecCaptureCadence/1(startIn), FEC Decoder Wrapper/2(startIn)
  dataIn/1 -> Automatic Gain Control/1(dataIn)
  Frequency and Time Synchronizer/1(dataOut) -> Bus Creator/3, QPSK Demodulator/1(dataIn), Delay4/1  "QPSKConstellationPoints"
  Automatic Gain Control/1(dataOut) -> RRC Receive Filter/1, Delay1/1
  Bus Creator/1 -> Delay/1
  Frequency and Time Synchronizer/7(nSynced) -> Bus Creator/1  "nSynced"
  RRC Receive Filter/2 -> Frequency and Time Synchronizer/2(validIn)
  Frequency and Time Synchronizer/3(endOut) -> QPSK Demodulator/3(endIn)
  Bus Creator1/1 -> ctrlOut/1
  Frequency and Time Synchronizer/8(normCoarseFreqEst) -> Bus Creator/2, CfcEstSI/1  "normCoarseFreqEst"
  RRC Receive Filter/1 -> Frequency and Time Synchronizer/1(dataIn)
  Automatic Gain Control/2(validOut) -> RRC Receive Filter/2
  validIn/1 -> Automatic Gain Control/2(validIn)
  rstCS/1 -> Frequency and Time Synchronizer/3(rstCS)
  FEC Decoder Wrapper/1(dataOut) -> dataOut/1
  FEC Decoder Wrapper/2(startOut) -> Bus Creator1/1
  FEC Decoder Wrapper/3(endOut) -> Bus Creator1/2
  FEC Decoder Wrapper/4(validOut) -> Bus Creator1/3
  FEC Decoder Wrapper/5(cnt_descr_in) -> cnt_descr_in/1
  FEC Decoder Wrapper/6(cnt_frame_start) -> cnt_frame_start/1
  FEC Decoder Wrapper/7(cnt_vit_reset) -> cnt_vit_reset/1
  FEC Decoder Wrapper/8(cnt_deint_valid) -> cnt_deint_valid/1
  FEC Decoder Wrapper/9(cnt_dec_bits) -> cnt_dec_bits/1
  FEC Decoder Wrapper/10(cnt_bist_start) -> cnt_bist_start/1
  skip_count/1 -> FEC Decoder Wrapper/5(skipCount)
  FEC Decoder Wrapper/11(cap_in) -> cap_in/1
  FEC Decoder Wrapper/12(cap_deint) -> cap_deint/1
  FEC Decoder Wrapper/13(cap_out) -> cap_out/1
  FecCaptureCadence/1(capCad) -> cap_cad/1
  QPSK Demodulator/1(dataOut) -> FEC Decoder Wrapper/1(bitsIn)
  QPSK Demodulator/3(endOut) -> FEC Decoder Wrapper/3(endIn)
  Frequency and Time Synchronizer/9(rstcsDet) -> RstCsCounter/1(e)
  CfcEstSI/1 -> CfcEstReg/1
  RstCsCounter/1(c) -> rstcs_count/1
  CfcEstReg/1 -> cfc_est/1
  Frequency and Time Synchronizer/10(p1c_telI) -> P1cToCplx/1
  Frequency and Time Synchronizer/11(p1c_telQ) -> P1cToCplx/2
  P1cToCplx/1 -> P1cDtc/1
  P1cDtc/1 -> Index Vector/6
  cs_prop_gain/1 -> Frequency and Time Synchronizer/4(cs_prop_gain)
  cs_integ_gain/1 -> Frequency and Time Synchronizer/5(cs_integ_gain)
  ss_prop_gain/1 -> Frequency and Time Synchronizer/6(ss_prop_gain)
  ss_integ_gain/1 -> Frequency and Time Synchronizer/7(ss_integ_gain)
  agc_loop_gain/1 -> Automatic Gain Control/3(agc_loop_gain)
  cfo_threshold/1 -> Frequency and Time Synchronizer/8(cfo_threshold)
  Frequency and Time Synchronizer/12(fs_runmax) -> fs_runmax/1

== system commhdlQPSKTxRxLoopback/TxRxComposite/Transmitter/Input Data ==
  enb : Inport
  reset : Inport  Port=2
  extWord : Inport  Port=3  OutDataTypeStr=uint64
  extWordAvail : Inport  Port=4  OutDataTypeStr=boolean
  extBitSel : Inport  Port=5  OutDataTypeStr=boolean
  extWordFirst : Inport  Port=6  OutDataTypeStr=boolean
  BitMux : Switch  Criteria=u2 ~= 0
  ByteBitShifter : MATLAB Function  TreatAsAtomicUnit=on
  Cast To Boolean : DataTypeConversion  OutDataTypeStr=boolean  SaturateOnIntegerOverflow=off  RndMeth=Floor
  Delay : Delay  DelayLength=1
  Display : Display
  FEC Tx Encoder K5 : Subsystem
  Message Generator : Subsystem
  Terminator : Terminator
  Terminator1 : Terminator
  txData : Outport
  txValid : Outport  Port=2
  msg_count_out : Outport  Port=3
  extWordPop : Outport  Port=4
  wires:
  Message Generator/6(msg_count_out) -> msg_count_out/1
  Message Generator/3(start) -> Terminator1/1, ByteBitShifter/3(start), FEC Tx Encoder K5/4(start)
  reset/1 -> Terminator/1
  Cast To Boolean/1 -> Message Generator/1(reset), ByteBitShifter/2(reset), FEC Tx Encoder K5/3(reset)
  Delay/1 -> Cast To Boolean/1
  Message Generator/2(stop) -> Delay/1
  Message Generator/5(count) -> Display/1
  enb/1 -> Message Generator/2(enable), ByteBitShifter/1(enable), FEC Tx Encoder K5/2(enable)
  Message Generator/4(valid) -> txValid/1
  extWord/1 -> ByteBitShifter/4(extWord)
  extWordAvail/1 -> ByteBitShifter/5(extWordAvail)
  extWordFirst/1 -> ByteBitShifter/6(extWordFirst)
  ByteBitShifter/2(popToggle) -> extWordPop/1
  extBitSel/1 -> BitMux/2
  Message Generator/1(out) -> BitMux/3
  BitMux/1 -> txData/1
  ByteBitShifter/1(bit) -> FEC Tx Encoder K5/1(bitIn)
  FEC Tx Encoder K5/1(encBit) -> BitMux/1

== system commhdlQPSKTxRxLoopback/TxRxComposite/Transmitter/QPSK Tx ==
  dataIn : Inport  OutDataTypeStr=boolean  PortDimensions=1
  validIn : Inport  Port=2  OutDataTypeStr=boolean  PortDimensions=1
  Bit Packetizer : Subsystem
  Bus Creator : BusCreator  Inputs=2
  HDL Data Scrambler : Subsystem
  QPSK Modulator : Subsystem
  RRC Transmit Filter : Subsystem
  dataReady : Outport
  dataOut : Outport  Port=2
  txDiagBus : Outport  Port=3
  validOut : Outport  Port=4
  wires:
  Bit Packetizer/4(bitsValid) -> HDL Data Scrambler/4(validIn)
  Bus Creator/1 -> txDiagBus/1
  Bit Packetizer/5(dataReady) -> dataReady/1
  Bit Packetizer/2(dataStart) -> HDL Data Scrambler/2(startIn)
  QPSK Modulator/1(dataOut) -> RRC Transmit Filter/1(dataIn), Bus Creator/1  "QPSKConstellationPoints"
  RRC Transmit Filter/1(dataOut) -> dataOut/1
  HDL Data Scrambler/2(validOut) -> QPSK Modulator/2(validIn)
  Bit Packetizer/3(dataEnd) -> HDL Data Scrambler/3(endIn)
  dataIn/1 -> Bit Packetizer/1(dataIn)
  QPSK Modulator/2(validOut) -> RRC Transmit Filter/2(validIn), Bus Creator/2  "QPSKConstellationValid"
  Bit Packetizer/1(bitsOut) -> HDL Data Scrambler/1(dataIn)
  HDL Data Scrambler/1(dataOut) -> QPSK Modulator/1(dataIn)
  RRC Transmit Filter/2(validOut) -> validOut/1
  validIn/1 -> Bit Packetizer/2(validIn)

== system commhdlQPSKTxRxLoopback/Receiver/QPSK Rx/Automatic Gain Control/Error Detector ==
  dataIn : Inport
  Add1 : Sum  Inputs=+-
  Conj : Math  Operator=conj
  Data Type Duplicate : DataTypeDuplicate
  Delay{,1..3} (4 alike) : Delay
  Product : Product
  Ref : Constant  Value=Ref  OutDataTypeStr=Inherit: Inherit via back propagation  SampleTime=-1
  err : Outport
  wires:
  Delay3/1 -> err/1
  Delay2/1 -> Add1/2
  Delay1/1 -> Product/1
  Delay/1 -> Product/2
  Ref/1 -> Data Type Duplicate/1, Add1/1
  Conj/1 -> Delay/1
  Product/1 -> Delay2/1
  dataIn/1 -> Conj/1, Data Type Duplicate/2, Delay1/1
  Add1/1 -> Delay3/1

== system commhdlQPSKTxRxLoopback/Receiver/QPSK Rx/Automatic Gain Control/Loop Filter ==
  note: Fixed point precision loss warnings
      | are supressed in Mask Init Callback
  err : Inport
  Add : Sum  Inputs=|++  OutDataTypeStr=Inherit: Same as first input
  Delay1 : Delay  DelayLength=1
  Delay2 : Delay
  Delay3 : Delay
  Gain1 : Gain  Gain=LFG  OutDataTypeStr=fixdt(1,34,28)
      mask init:
      | Simulink.suppressDiagnostic(gcb, 'SimulinkFixedPoint:util:fxpParameterPrecisionLoss');
  gain : Outport
  wires:
  Delay3/1 -> Gain1/1
  Delay2/1 -> Add/1
  Gain1/1 -> Delay2/1
  Add/1 -> Delay1/1
  Delay1/1 -> Add/2, gain/1
  err/1 -> Delay3/1

== system commhdlQPSKTxRxLoopback/Receiver/QPSK Rx/Frequency and Time Synchronizer/Carrier Synchronizer ==
  dataIn : Inport
  internalRst : Inport  Port=2
  validIn : Inport  Port=3
  manualRst : Inport  Port=4
  Data Type Conversion2 : DataTypeConversion  OutDataTypeStr=fixdt(1,16,14)  SaturateOnIntegerOverflow=off  RndMeth=Floor
  Delay{,2,5,7,11} (5 alike) : Delay  DelayLength=1
  Delay{1,10,14..15} (4 alike) : Delay  DelayLength=6
  Delay{3..4,6,8..9,12..13} (7 alike) : Delay
  Direct Digital Synthesis : Subsystem
  Logical Operator : Logic  AllPortsSameDT=off  OutDataTypeStr=boolean
  Loop Filter : Subsystem
  Math Function : Math  Operator=conj  SignedPower=on  RndMeth=Zero
  Phase Error Detector : Subsystem
  Product : Product
  dataOut : Outport
  validOut : Outport  Port=2
  wires:
  Delay/1 -> Phase Error Detector/1(dataIn)
  Math Function/1 -> Delay3/1
  Data Type Conversion2/1 -> Delay5/1, Delay/1
  Delay3/1 -> Product/2
  Product/1 -> Delay6/1
  Delay8/1 -> Delay2/1, Delay7/1
  Delay9/1 -> Delay8/1
  Delay4/1 -> Product/1
  Delay6/1 -> Data Type Conversion2/1
  Direct Digital Synthesis/1(expOut) -> Math Function/1
  Loop Filter/1(v) -> Direct Digital Synthesis/3(phaseInc)
  Phase Error Detector/1(PhaseError) -> Loop Filter/1(e)
  Delay2/1 -> Delay1/1
  Delay1/1 -> Loop Filter/2(validIn)
  Delay10/1 -> Delay4/1
  Delay11/1 -> Delay15/1
  Delay12/1 -> Delay11/1
  Delay13/1 -> Delay12/1
  Loop Filter/2(valid) -> Direct Digital Synthesis/2(validIn)
  Delay5/1 -> dataOut/1
  Delay7/1 -> validOut/1
  dataIn/1 -> Delay10/1
  internalRst/1 -> Delay13/1
  validIn/1 -> Delay14/1
  Delay14/1 -> Delay9/1
  manualRst/1 -> Logical Operator/1, Loop Filter/4(externalRst)
  Delay15/1 -> Loop Filter/3(internalRst)
  Loop Filter/3(rst) -> Logical Operator/2
  Logical Operator/1 -> Direct Digital Synthesis/1(rst)
